simulink model "INS"  (R2018b)
settings: configuration reference "ins_config" (kept outside this file)
values from neighbouring files (symbols this model uses):
  INS_EXPORT = Simulink.Parameter(INS_EXPORT_VALUE)    [ins_model_init.m]
  INS_PARAM = Simulink.Parameter(INS_PARAM_VALUE)    [ins_model_init.m]
undefined symbols (not defined in the file or in its folder): DiscIntNeverNeededParam, INS_CONST, INS_EXPORT_VALUE, Sensor_Meas
libraries: simulink x131, FMT_Model_Lib x48
(part 2 of 6)

== system INS/Sensor_PreProcess/MAG_PreProcess/Mag_Data_Process ==
  mag_B_uT : Inport
  mag_valid : Inport  Port=2
  DCM_OB : Inport  Port=3
  GPS_Data : Inport  Port=4
  Bus Selector : BusSelector  OutputSignals=lat_0_rad,lon_0_rad
  Bus Selector1 : BusSelector  OutputSignals=GPS_valid
  Mag_Quality_Estimate : Subsystem
  WMM_Compensation : Subsystem
  WMM_LUT : Subsystem  mask{wmm_magnitude=INS_CONST.wmm_mag, wmm_declination=INS_CONST.wmm_dec, wmm_inclination=INS_CONST.wmm_inc, resolution=10}
      mask prompts: wmm_magnitude "WMM Magnitude Lookup Table"; wmm_declination "WMM Declination Lookup Table"; wmm_inclination "WMM Inclination Lookup Table"; resolution "Resolution (deg)"
  mag_normalized_B : Outport
  mag_quality : Outport  Port=2
  wires:
  Mag_Quality_Estimate/1(mag_quality) -> mag_quality/1
  WMM_LUT/3(inclination_deg) -> Mag_Quality_Estimate/2(nominal_inc_deg)
  mag_B_uT/1 -> WMM_Compensation/4(mag_B_uT)
  DCM_OB/1 -> WMM_Compensation/3(DCM_OB)
  WMM_Compensation/2(mag_normalized_O) -> Mag_Quality_Estimate/1(mag_normalized_O)
  WMM_LUT/1(magnitude_uT) -> WMM_Compensation/1(WMM_magnitude_uT)
  WMM_LUT/2(declination_deg) -> WMM_Compensation/2(WMM_declination_deg)
  GPS_Data/1 -> Bus Selector1/1, Bus Selector/1
  Bus Selector/1 -> WMM_LUT/1(lat_rad)  "<lat_0_rad>"
  Bus Selector/2 -> WMM_LUT/2(lon_rad)  "<lon_0_rad>"
  Bus Selector1/1 -> Mag_Quality_Estimate/3(pos_0_valid), WMM_Compensation/5(pos_0_valid)  "<GPS_valid>"
  mag_valid/1 -> Mag_Quality_Estimate/4(mag_valid)
  WMM_Compensation/1(mag_normalized_B) -> mag_normalized_B/1

== system INS/Sensor_PreProcess/MAG_PreProcess/Sensor_Valid ==
  mag_B_gauss : Inport
  timestamp_ms : Inport  Port=2
  Compare To Constant4 : simulink/Logic and Bit Operations/Compare To Constant  relop=<  const=timeout  OutDataTypeStr=boolean
  Constant : Constant  Value=INS_EXPORT.period  OutDataTypeStr=single
  Detect Change : simulink/Logic and Bit Operations/Detect Change  vinit=0  OutDataTypeStr=boolean
  Discrete-Time Integrator : DiscreteIntegrator  IntegratorMethod=Accumulation: Forward Euler  ExternalReset=sampled level  SampleTime=-1  OutDataTypeStr=uint32  SaturateOnIntegerOverflow=on  ICPrevOutput=DiscIntNeverNeededParam  ICPrevScaledInput=DiscIntNeverNeededParam
  Ever_Valid : Subsystem
  Interval Test1 : simulink/Logic and Bit Operations/Interval Test  IntervalClosedRight=off  uplimit=mag_max  IntervalClosedLeft=off  lowlimit=mag_min  OutDataTypeStr=boolean
  Logical Operator1 : Logic  Inputs=1  AllPortsSameDT=off  OutDataTypeStr=boolean
  Logical Operator4 : Logic  Inputs=3  AllPortsSameDT=off  OutDataTypeStr=boolean
  valid : Outport
  wires:
  Logical Operator4/1 -> valid/1
  Compare To Constant4/1 -> Logical Operator4/2
  Discrete-Time Integrator/1 -> Compare To Constant4/1
  Detect Change/1 -> Ever_Valid/1(in), Discrete-Time Integrator/2
  Constant/1 -> Discrete-Time Integrator/1
  Logical Operator1/1 -> Logical Operator4/1
  timestamp_ms/1 -> Detect Change/1
  mag_B_gauss/1 -> Interval Test1/1
  Interval Test1/1 -> Logical Operator1/1
  Ever_Valid/1(out) -> Logical Operator4/3

== system INS/Sensor_PreProcess/OpticalFlow_PreProcess/Height_Compensation ==
  OpticalFlow_Bus : Inport
  IMU_Data : Inport  Port=2
  Rangefinder_Data : Inport  Port=3
  Bus Selector : BusSelector  OutputSignals=vx,vy
  Bus Selector1 : BusSelector  OutputSignals=distance,valid
  Bus Selector2 : BusSelector  OutputSignals=gyr_y,gyr_x
  DeadZone : Subsystem  mask{dz=0.5}
      mask prompts: dz "dead zone"
  Demux : Demux  Outputs=2
  First Order LPF : FMT_Model_Lib/Filter/First Order LPF  fc=30
      settings: SourceProductName=FMT Toolbox
  First Order LPF1 : FMT_Model_Lib/Filter/First Order LPF  fc=10
      settings: SourceProductName=FMT Toolbox
  Gain : Gain  Gain=-1
  Gain1 : Gain  Gain=INS_PARAM.OPF_FIX_GAIN
  Multiply : Product  Inputs=3
  Mux : Mux  Inputs=2
  Mux1 : Mux  Inputs=2
  Sum : Sum  Inputs=|+-
  vx_B_mPs : Outport
  vy_B_mPs : Outport  Port=2
  wires:
  Rangefinder_Data/1 -> Bus Selector1/1
  OpticalFlow_Bus/1 -> Bus Selector/1
  Bus Selector/1 -> Mux/1  "<vx>"
  Bus Selector/2 -> Mux/2  "<vy>"
  Bus Selector1/1 -> Multiply/2  "<distance>"
  Mux/1 -> First Order LPF/1
  Demux/1 -> vx_B_mPs/1
  Demux/2 -> vy_B_mPs/1
  First Order LPF/1 -> Sum/1  "raw_vxy"
  Multiply/1 -> Demux/1
  Bus Selector1/2 -> Multiply/3  "<valid>"
  IMU_Data/1 -> Bus Selector2/1
  Bus Selector2/1 -> Mux1/1  "<gyr_y>"
  Bus Selector2/2 -> Gain/1  "<gyr_x>"
  Gain/1 -> Mux1/2
  Mux1/1 -> First Order LPF1/1
  DeadZone/1(y) -> Gain1/1
  Gain1/1 -> Sum/2  "gyro_vxy"
  Sum/1 -> Multiply/1  "fix_vxy"
  First Order LPF1/1 -> DeadZone/1(u)

== system INS/Sensor_PreProcess/OpticalFlow_PreProcess/Sensor_Valid ==
  OpticalFlow_Bus : Inport
  Rangefinder_Data : Inport  Port=2
  Bus Selector : BusSelector  OutputSignals=vx,vy,quality,timestamp
  Bus Selector1 : BusSelector  OutputSignals=valid
  Compare To Constant4 : simulink/Logic and Bit Operations/Compare To Constant  relop=<  const=timeout  OutDataTypeStr=boolean
  Constant : Constant  Value=INS_EXPORT.period  OutDataTypeStr=single
  Detect Change : simulink/Logic and Bit Operations/Detect Change  vinit=0  OutDataTypeStr=boolean
  Discrete-Time Integrator : DiscreteIntegrator  IntegratorMethod=Accumulation: Forward Euler  ExternalReset=sampled level  SampleTime=-1  OutDataTypeStr=uint32  SaturateOnIntegerOverflow=on  ICPrevOutput=DiscIntNeverNeededParam  ICPrevScaledInput=DiscIntNeverNeededParam
  Ever_Valid : Subsystem
  Interval Test1 : simulink/Logic and Bit Operations/Interval Test  IntervalClosedRight=off  uplimit=max_vel  IntervalClosedLeft=off  lowlimit=min_vel  OutDataTypeStr=boolean
  Interval Test2 : simulink/Logic and Bit Operations/Interval Test  IntervalClosedRight=off  uplimit=max_vel  IntervalClosedLeft=off  lowlimit=min_vel  OutDataTypeStr=boolean
  Logical Operator : Logic  AllPortsSameDT=off  OutDataTypeStr=boolean
  Logical Operator1 : Logic  Inputs=5  AllPortsSameDT=off  OutDataTypeStr=boolean
  Relay : Relay  OnOutputValue=q_high  OffOutputValue=q_low
  valid : Outport
  wires:
  Logical Operator1/1 -> valid/1
  Compare To Constant4/1 -> Logical Operator1/3
  Detect Change/1 -> Ever_Valid/1(in), Discrete-Time Integrator/2
  Constant/1 -> Discrete-Time Integrator/1
  Discrete-Time Integrator/1 -> Compare To Constant4/1
  Bus Selector/4 -> Detect Change/1  "<timestamp>"
  OpticalFlow_Bus/1 -> Bus Selector/1
  Bus Selector/1 -> Interval Test1/1  "<vx>"
  Bus Selector/2 -> Interval Test2/1  "<vy>"
  Interval Test1/1 -> Logical Operator/1
  Interval Test2/1 -> Logical Operator/2
  Bus Selector/3 -> Relay/1  "<quality>"
  Logical Operator/1 -> Logical Operator1/1
  Relay/1 -> Logical Operator1/2
  Rangefinder_Data/1 -> Bus Selector1/1
  Bus Selector1/1 -> Logical Operator1/5  "<valid>"
  Ever_Valid/1(out) -> Logical Operator1/4

== system INS/Sensor_PreProcess/Rangefinder_PreProcess/Sensor_Valid ==
  Rangefinder_Bus : Inport
  Bus Selector : BusSelector  OutputSignals=distance,timestamp
  Compare To Constant4 : simulink/Logic and Bit Operations/Compare To Constant  relop=<  const=timeout  OutDataTypeStr=boolean
  Constant : Constant  Value=INS_EXPORT.period  OutDataTypeStr=single
  Detect Change : simulink/Logic and Bit Operations/Detect Change  vinit=0  OutDataTypeStr=boolean
  Discrete-Time Integrator : DiscreteIntegrator  IntegratorMethod=Accumulation: Forward Euler  ExternalReset=sampled level  SampleTime=-1  OutDataTypeStr=uint32  SaturateOnIntegerOverflow=on  ICPrevOutput=DiscIntNeverNeededParam  ICPrevScaledInput=DiscIntNeverNeededParam
  Ever_Valid : Subsystem
  Interval Test3 : simulink/Logic and Bit Operations/Interval Test  IntervalClosedRight=off  uplimit=max_alt  IntervalClosedLeft=off  lowlimit=min_alt  OutDataTypeStr=boolean
  Logical Operator1 : Logic  Inputs=4  AllPortsSameDT=off  OutDataTypeStr=boolean
  Relay : Relay  OnSwitchValue=max_alt  OffSwitchValue=max_alt-(max_alt-min_alt)/4  OnOutputValue=0  OffOutputValue=1
  valid : Outport
  wires:
  Bus Selector/1 -> Interval Test3/1, Relay/1  "<distance>"
  Rangefinder_Bus/1 -> Bus Selector/1
  Bus Selector/2 -> Detect Change/1  "<timestamp>"
  Discrete-Time Integrator/1 -> Compare To Constant4/1
  Constant/1 -> Discrete-Time Integrator/1
  Relay/1 -> Logical Operator1/2
  Compare To Constant4/1 -> Logical Operator1/3
  Logical Operator1/1 -> valid/1
  Detect Change/1 -> Ever_Valid/1(in), Discrete-Time Integrator/2
  Ever_Valid/1(out) -> Logical Operator1/4
  Interval Test3/1 -> Logical Operator1/1

== system INS/Sensor_PreProcess/Rangefinder_PreProcess/Subsystem ==
  in : Inport
  Compare To Constant : simulink/Logic and Bit Operations/Compare To Constant  relop=>=  const=20  OutDataTypeStr=boolean
  Compare To Zero : simulink/Logic and Bit Operations/Compare To Zero  relop=>  OutDataTypeStr=boolean
  Discrete-Time Integrator : DiscreteIntegrator  IntegratorMethod=Accumulation: Forward Euler  ExternalReset=falling  SampleTime=-1  OutDataTypeStr=uint32  LimitOutput=on  UpperSaturationLimit=9999  LowerSaturationLimit=0  ICPrevOutput=DiscIntNeverNeededParam  ICPrevScaledInput=DiscIntNeverNeededParam
  out : Outport
  wires:
  in/1 -> Compare To Zero/1
  Compare To Zero/1 -> Discrete-Time Integrator/2, Discrete-Time Integrator/1
  Discrete-Time Integrator/1 -> Compare To Constant/1
  Compare To Constant/1 -> out/1

== system INS/Sensor_PreProcess/Rangefinder_PreProcess/Tilt_Compensation ==
  Rangefinder_Bus : Inport
  Rotation_Data : Inport  Port=2
  Bus Selector : BusSelector  OutputSignals=distance
  Bus Selector1 : BusSelector  OutputSignals=phi_rad,theta_rad
  Cos : Trigonometry  Operator=cos
  Cos1 : Trigonometry  Operator=cos
  Multiply : Product  Inputs=3
  raw_distance : Outport
  distance : Outport  Port=2
  wires:
  Bus Selector1/1 -> Cos/1  "<phi_rad>"
  Cos/1 -> Multiply/2
  Rangefinder_Bus/1 -> Bus Selector/1
  Multiply/1 -> distance/1
  Bus Selector/1 -> raw_distance/1, Multiply/1  "<distance>"
  Bus Selector1/2 -> Cos1/1  "<theta_rad>"
  Cos1/1 -> Multiply/3
  Rotation_Data/1 -> Bus Selector1/1

== system INS/Bus_Constructor/Status_Output/INS_Flag/INS_Ready ==
  Rotation_Data : Inport
  Bus Selector : BusSelector  OutputSignals=att_reset,heading_reset
  Delay : Delay  DelayLength=1
  Delay1 : Delay  DelayLength=1
  Detect Increase : simulink/Logic and Bit Operations/Detect Increase  vinit=0.0  OutDataTypeStr=boolean
  Detect Increase1 : simulink/Logic and Bit Operations/Detect Increase  vinit=0.0  OutDataTypeStr=boolean
  Logical Operator : Logic  AllPortsSameDT=off  OutDataTypeStr=boolean
  Logical Operator1 : Logic  Operator=OR  AllPortsSameDT=off  OutDataTypeStr=boolean
  Logical Operator2 : Logic  Operator=OR  AllPortsSameDT=off  OutDataTypeStr=boolean
  ready : Outport
  wires:
  Rotation_Data/1 -> Bus Selector/1
  Detect Increase/1 -> Logical Operator1/1
  Logical Operator1/1 -> Logical Operator/1, Delay/1
  Delay/1 -> Logical Operator1/2
  Bus Selector/1 -> Detect Increase/1  "<att_reset>"
  Logical Operator2/1 -> Logical Operator/2, Delay1/1
  Detect Increase1/1 -> Logical Operator2/1
  Delay1/1 -> Logical Operator2/2
  Bus Selector/2 -> Detect Increase1/1  "<heading_reset>"
  Logical Operator/1 -> ready/1

== system INS/Bus_Constructor/Status_Output/INS_Flag/valid_check5 ==
  quality : Inport
  Compare To Constant : simulink/Logic and Bit Operations/Compare To Constant  relop=>=  const=time_out  OutDataTypeStr=boolean
  Compare To Constant1 : simulink/Logic and Bit Operations/Compare To Constant  relop=>  const=0  OutDataTypeStr=boolean
  Compare To Constant2 : simulink/Logic and Bit Operations/Compare To Constant  relop=>  const=0  OutDataTypeStr=boolean
  Constant : Constant  Value=INS_EXPORT.period  OutDataTypeStr=Inherit: Inherit via back propagation
  Delay : Delay  DelayLength=1
  Detect Rise Positive : simulink/Logic and Bit Operations/Detect Rise Positive  vinit=0  OutDataTypeStr=boolean
  Discrete-Time Integrator : DiscreteIntegrator  IntegratorMethod=Accumulation: Forward Euler  gainval=1  ExternalReset=level  SampleTime=-1  LimitOutput=on  UpperSaturationLimit=1e6  LowerSaturationLimit=0  ICPrevOutput=DiscIntNeverNeededParam  ICPrevScaledInput=DiscIntNeverNeededParam
  Logical Operator : Logic  Operator=NOT  AllPortsSameDT=off  OutDataTypeStr=boolean
  Logical Operator1 : Logic  Operator=OR  AllPortsSameDT=off  OutDataTypeStr=boolean
  Multiply : Product
  valid : Outport
  wires:
  Multiply/1 -> valid/1
  Delay/1 -> Multiply/2, Logical Operator1/2
  Logical Operator1/1 -> Delay/1
  Detect Rise Positive/1 -> Logical Operator1/1
  Compare To Constant2/1 -> Detect Rise Positive/1
  quality/1 -> Compare To Constant1/1, Compare To Constant2/1
  Compare To Constant1/1 -> Discrete-Time Integrator/2
  Constant/1 -> Discrete-Time Integrator/1
  Discrete-Time Integrator/1 -> Compare To Constant/1
  Compare To Constant/1 -> Logical Operator/1
  Logical Operator/1 -> Multiply/1

== system INS/Bus_Constructor/Status_Output/INS_Flag/valid_check8 ==
  quality : Inport
  Compare To Constant : simulink/Logic and Bit Operations/Compare To Constant  relop=>=  const=time_out  OutDataTypeStr=boolean
  Compare To Constant1 : simulink/Logic and Bit Operations/Compare To Constant  relop=>  const=0  OutDataTypeStr=boolean
  Compare To Constant2 : simulink/Logic and Bit Operations/Compare To Constant  relop=>  const=0  OutDataTypeStr=boolean
  Constant : Constant  Value=INS_EXPORT.period  OutDataTypeStr=Inherit: Inherit via back propagation
  Delay : Delay  DelayLength=1
  Detect Rise Positive : simulink/Logic and Bit Operations/Detect Rise Positive  vinit=0  OutDataTypeStr=boolean
  Discrete-Time Integrator : DiscreteIntegrator  IntegratorMethod=Accumulation: Forward Euler  gainval=1  ExternalReset=level  SampleTime=-1  LimitOutput=on  UpperSaturationLimit=1e6  LowerSaturationLimit=0  ICPrevOutput=DiscIntNeverNeededParam  ICPrevScaledInput=DiscIntNeverNeededParam
  Logical Operator : Logic  Operator=NOT  AllPortsSameDT=off  OutDataTypeStr=boolean
  Logical Operator1 : Logic  Operator=OR  AllPortsSameDT=off  OutDataTypeStr=boolean
  Multiply : Product
  valid : Outport
  wires:
  Multiply/1 -> valid/1
  Delay/1 -> Multiply/2, Logical Operator1/2
  Logical Operator1/1 -> Delay/1
  Detect Rise Positive/1 -> Logical Operator1/1
  Compare To Constant2/1 -> Detect Rise Positive/1
  quality/1 -> Compare To Constant1/1, Compare To Constant2/1
  Compare To Constant1/1 -> Discrete-Time Integrator/2
  Constant/1 -> Discrete-Time Integrator/1
  Discrete-Time Integrator/1 -> Compare To Constant/1
  Compare To Constant/1 -> Logical Operator/1
  Logical Operator/1 -> Multiply/1

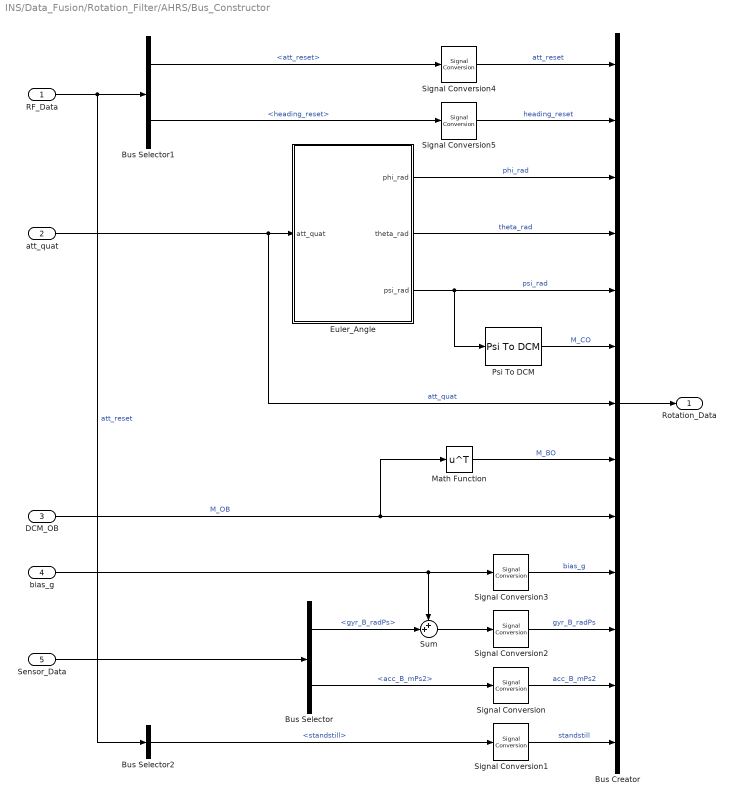
== system INS/Data_Fusion/Rotation_Filter/AHRS/Bus_Constructor ==
  RF_Data : Inport
  att_quat : Inport  Port=2
  DCM_OB : Inport  Port=3
  bias_g : Inport  Port=4
  Sensor_Data : Inport  Port=5
  Bus Creator : BusCreator  Inputs=13
  Bus Selector : BusSelector  OutputSignals=IMU_Data.gyr_B_radPs,IMU_Data.acc_B_mPs2
  Bus Selector1 : BusSelector  OutputSignals=att_reset,heading_reset
  Bus Selector2 : BusSelector  OutputSignals=standstill
  Euler_Angle : Subsystem
  Math Function : Math  Operator=transpose  SaturateOnIntegerOverflow=on
  Psi To DCM : FMT_Model_Lib/Transformation/Psi To DCM
      settings: SourceProductName=FMT Toolbox
  Signal Conversion{,1..5} (6 alike) : SignalConversion  OverrideOpt=off
  Sum : Sum  Inputs=++|
  Rotation_Data : Outport
  wires:
  Bus Selector1/1 -> Signal Conversion4/1  "<att_reset>"
  Signal Conversion/1 -> Bus Creator/12  "acc_B_mPs2"
  Euler_Angle/1(phi_rad) -> Bus Creator/3  "phi_rad"
  Euler_Angle/2(theta_rad) -> Bus Creator/4  "theta_rad"
  Euler_Angle/3(psi_rad) -> Psi To DCM/1, Bus Creator/5  "psi_rad"
  Sensor_Data/1 -> Bus Selector/1
  Bus Selector2/1 -> Signal Conversion1/1  "<standstill>"
  Bus Creator/1 -> Rotation_Data/1
  bias_g/1 -> Sum/1, Signal Conversion3/1
  Math Function/1 -> Bus Creator/8  "M_BO"
  DCM_OB/1 -> Math Function/1, Bus Creator/9  "M_OB"
  att_quat/1 -> Euler_Angle/1(att_quat), Bus Creator/7  "att_quat"
  Psi To DCM/1 -> Bus Creator/6  "M_CO"
  Signal Conversion1/1 -> Bus Creator/13  "standstill"
  Bus Selector/2 -> Signal Conversion/1  "<acc_B_mPs2>"
  Signal Conversion2/1 -> Bus Creator/11  "gyr_B_radPs"
  Signal Conversion3/1 -> Bus Creator/10  "bias_g"
  RF_Data/1 -> Bus Selector2/1, Bus Selector1/1  "att_reset"
  Bus Selector/1 -> Sum/2  "<gyr_B_radPs>"
  Signal Conversion4/1 -> Bus Creator/1  "att_reset"
  Bus Selector1/2 -> Signal Conversion5/1  "<heading_reset>"
  Signal Conversion5/1 -> Bus Creator/2  "heading_reset"
  Sum/1 -> Signal Conversion2/1

== system INS/Data_Fusion/Rotation_Filter/AHRS/Correct ==
  Rotation_Data : Inport
  Translation_Data : Inport  Port=2
  Sensor_Data : Inport  Port=3
  RF_Data : Inport  Port=4
  Attitude_Correction : Subsystem
  Bus Selector1 : BusSelector  OutputSignals=IMU_Data
  Gyro_Bias_Correction : Subsystem
  att_B_correction : Outport
  bias_g_B_correction : Outport  Port=2
  wires:
  Gyro_Bias_Correction/1(bias_g_B_correction) -> bias_g_B_correction/1
  Bus Selector1/1 -> Gyro_Bias_Correction/2(IMU_Data)  "<IMU_Data>"
  RF_Data/1 -> Attitude_Correction/4(RF_Data)
  Attitude_Correction/1(att_B_correction) -> att_B_correction/1, Gyro_Bias_Correction/1(att_B_correction)
  Sensor_Data/1 -> Attitude_Correction/2(Sensor_Data), Bus Selector1/1
  Rotation_Data/1 -> Attitude_Correction/3(Rotation_Data)
  Translation_Data/1 -> Attitude_Correction/1(Translation_Data)

== system INS/Data_Fusion/Rotation_Filter/AHRS/Update ==
  att_B_correction : Inport
  bias_g_correction : Inport  Port=2
  RF_Data : Inport  Port=3
  Sensor_Data : Inport  Port=4
  Attitude_Update : Subsystem
  Attitude_Update1 : Subsystem  Commented=on
  Bus Selector : BusSelector  OutputSignals=IMU_Data.gyr_B_radPs
  Bus Selector1 : BusSelector  OutputSignals=att_reset,quat_0
  Gyro_Bias_Update : Subsystem
  Sum2 : Sum  Inputs=|++
  att_quat : Outport
  DCM_OB : Outport  Port=2
  bias_g : Outport  Port=3
  wires:
  Sensor_Data/1 -> Bus Selector/1
  Gyro_Bias_Update/1(gyr_B_correction) -> Sum2/2
  att_B_correction/1 -> Sum2/1
  Sum2/1 -> Attitude_Update/3(att_B_correction)
  Bus Selector/1 -> Gyro_Bias_Update/2(gyr_B_radPs)  "<gyr_B_radPs>"
  bias_g_correction/1 -> Gyro_Bias_Update/1(bias_g_correction)
  Attitude_Update/1(att_quat) -> att_quat/1
  Attitude_Update/2(DCM_OB) -> DCM_OB/1
  Gyro_Bias_Update/2(bias_g) -> bias_g/1
  RF_Data/1 -> Bus Selector1/1  "att_reset"
  Bus Selector1/1 -> Attitude_Update/1(att_reset)  "<att_reset>"
  Bus Selector1/2 -> Attitude_Update/2(quat_0)  "<quat_0>"

== system INS/Data_Fusion/Rotation_Filter/RF_Data_PreProcess/Attitude_Reset ==
  Sensor_Data : Inport
  Bus Selector : BusSelector  OutputSignals=IMU_Data.IMU_valid,IMU_Data.acc_B_mPs2
  Bus Selector2 : BusSelector  OutputSignals=Mag_Data.mag_quality,Mag_Data.mag_norm_B
  Bus Selector3 : BusSelector  OutputSignals=ExternalPos_Data.heading_valid,GPS_Data.heading_valid
  Compare To Constant : simulink/Logic and Bit Operations/Compare To Constant  relop=>  const=0.01  OutDataTypeStr=boolean
  Compare To Constant1 : simulink/Logic and Bit Operations/Compare To Constant  relop=>=  const=0.2  OutDataTypeStr=boolean
  Detect Rise Positive : simulink/Logic and Bit Operations/Detect Rise Positive  vinit=0  OutDataTypeStr=boolean
  Detect Rise Positive1 : simulink/Logic and Bit Operations/Detect Rise Positive  vinit=0  OutDataTypeStr=boolean
  Interval Test : simulink/Logic and Bit Operations/Interval Test  IntervalClosedRight=on  uplimit=INS_CONST.g+0.5  IntervalClosedLeft=on  lowlimit=INS_CONST.g-0.5  OutDataTypeStr=boolean
  Logical Operator1 : Logic  AllPortsSameDT=off  OutDataTypeStr=boolean
  Logical Operator3 : Logic  AllPortsSameDT=off  OutDataTypeStr=boolean
  Logical Operator4 : Logic  Operator=OR  Inputs=3  AllPortsSameDT=off  OutDataTypeStr=boolean
  Logical Operator5 : Logic  Operator=OR  AllPortsSameDT=off  OutDataTypeStr=boolean
  Vector Modulus : FMT_Model_Lib/Math/Vector Modulus
      settings: SourceProductName=FMT Toolbox
  Vector Modulus1 : FMT_Model_Lib/Math/Vector Modulus
      settings: SourceProductName=FMT Toolbox
  sample_valid : Subsystem
  sample_valid1 : Subsystem
  att_reset : Outport
  heading_reset : Outport  Port=2
  wires:
  sample_valid/1(imu_valid) -> Detect Rise Positive/1  "tt2"
  Vector Modulus1/1 -> Compare To Constant/1
  Interval Test/1 -> Logical Operator1/2
  Vector Modulus/1 -> Interval Test/1
  Logical Operator1/1 -> sample_valid/1(valid)
  Sensor_Data/1 -> Bus Selector2/1, Bus Selector3/1, Bus Selector/1
  Bus Selector/2 -> Vector Modulus/1  "<acc_B_mPs2>"
  Bus Selector/1 -> Logical Operator1/1  "<IMU_valid>"
  Bus Selector2/2 -> Vector Modulus1/1  "<mag_norm_B>"
  Bus Selector2/1 -> Compare To Constant1/1  "<mag_quality>"
  Compare To Constant/1 -> Logical Operator3/2
  Compare To Constant1/1 -> Logical Operator3/1
  Logical Operator3/1 -> sample_valid1/1(valid)
  sample_valid1/1(mag_valid) -> Logical Operator4/1  "tt1"
  Bus Selector3/1 -> Logical Operator4/2  "<heading_valid>"
  Logical Operator4/1 -> Detect Rise Positive1/1
  Detect Rise Positive1/1 -> Logical Operator5/2, heading_reset/1
  Detect Rise Positive/1 -> Logical Operator5/1
  Logical Operator5/1 -> att_reset/1
  Bus Selector3/2 -> Logical Operator4/3  "<heading_valid>"

== system INS/Data_Fusion/Rotation_Filter/RF_Data_PreProcess/Initial_Attitude ==
  Sensor_Data : Inport
  Enable : EnablePort
  Bus Selector : BusSelector  OutputSignals=IMU_Data.acc_B_mPs2
  Cross Product : FMT_Model_Lib/Math/Cross Product
      settings: SourceProductName=FMT Toolbox
  Cross Product1 : FMT_Model_Lib/Math/Cross Product
      settings: SourceProductName=FMT Toolbox
  DCM To Quaternion : FMT_Model_Lib/Quaternion/DCM To Quaternion
      settings: SourceProductName=FMT Toolbox
  Gain : Gain  Gain=-1
  Heading_Vector : Subsystem
  Vector Concatenate : Concatenate  NumInputs=3  Mode=Multidimensional array  ConcatenateDimension=2
  Vector Normalize : FMT_Model_Lib/Math/Vector Normalize
      settings: SourceProductName=FMT Toolbox
  Vector Normalize1 : FMT_Model_Lib/Math/Vector Normalize
      settings: SourceProductName=FMT Toolbox
  Vector Normalize2 : FMT_Model_Lib/Math/Vector Normalize
      settings: SourceProductName=FMT Toolbox
  quat_0 : Outport  InitialOutput=[1; 0; 0; 0]
  wires:
  Gain/1 -> Cross Product/1, Vector Normalize2/1, Cross Product1/2
  Cross Product1/1 -> Vector Normalize/1
  Cross Product/1 -> Vector Normalize1/1, Cross Product1/1
  Vector Normalize1/1 -> Vector Concatenate/2  "DCM_y"
  Vector Normalize/1 -> Vector Concatenate/1  "DCM_x"
  Vector Normalize2/1 -> Vector Concatenate/3  "DCM_z"
  DCM To Quaternion/1 -> quat_0/1
  Sensor_Data/1 -> Bus Selector/1, Heading_Vector/1(Sensor_Data)
  Bus Selector/1 -> Gain/1  "<acc_B_mPs2>"
  Vector Concatenate/1 -> DCM To Quaternion/1  "M_BO"
  Heading_Vector/1(heading_vec) -> Cross Product/2

== system INS/Data_Fusion/Rotation_Filter/RF_Data_PreProcess/Sensor_Select ==
  standstill : Inport
  Sensor_Data : Inport  Port=2
  Bus Selector : BusSelector  OutputSignals=ExternalPos_Data.heading_valid,GPS_Data.heading_valid
  Bus Selector1 : BusSelector  OutputSignals=Mag_Data.mag_valid
  Constant1 : Constant  Value=INS_PARAM.MAG_FLY_EN
  Logical Operator1 : Logic  Operator=NOT  AllPortsSameDT=off  OutDataTypeStr=boolean
  Logical Operator2 : Logic  AllPortsSameDT=off  OutDataTypeStr=boolean
  Logical Operator3 : Logic  Operator=NOT  AllPortsSameDT=off  OutDataTypeStr=boolean
  Logical Operator4 : Logic  Operator=OR  AllPortsSameDT=off  OutDataTypeStr=boolean
  Logical Operator5 : Logic  Inputs=4  AllPortsSameDT=off  OutDataTypeStr=boolean
  ext_psi_enable : Outport
  gps_psi_enable : Outport  Port=2
  mag_enable : Outport  Port=3
  wires:
  Sensor_Data/1 -> Bus Selector/1, Bus Selector1/1
  Bus Selector/1 -> ext_psi_enable/1, Logical Operator3/1  "<heading_valid>"
  Bus Selector1/1 -> Logical Operator5/3  "<mag_valid>"
  Constant1/1 -> Logical Operator4/1
  standstill/1 -> Logical Operator4/2
  Logical Operator5/1 -> mag_enable/1
  Logical Operator3/1 -> Logical Operator2/1, Logical Operator5/1
  Logical Operator4/1 -> Logical Operator5/4
  Logical Operator1/1 -> Logical Operator5/2
  Logical Operator2/1 -> gps_psi_enable/1
  Bus Selector/2 -> Logical Operator1/1, Logical Operator2/2  "<heading_valid>"

== system INS/Data_Fusion/Rotation_Filter/RF_Data_PreProcess/Standstill ==
  IMU_Data : Inport
  Abs : Abs
  Bus Selector : BusSelector  OutputSignals=gyr_B_radPs
  First Order HPF : FMT_Model_Lib/Filter/First Order HPF  fc=1/(2*pi*0.2)
      settings: SourceProductName=FMT Toolbox
  First Order LPF : FMT_Model_Lib/Filter/First Order LPF  fc=1/(2*pi*0.1)
      settings: SourceProductName=FMT Toolbox
  First Order LPF1 : FMT_Model_Lib/Filter/First Order LPF  fc=1/(2*pi*0.05)
      settings: SourceProductName=FMT Toolbox
  MinMax1 : MinMax  Function=max
  Relay : Relay  OnSwitchValue=10e-3  OffSwitchValue=4e-3  OnOutputValue=0  OffOutputValue=1
  Saturation2 : Saturate  UpperLimit=1  LowerLimit=0
  Selector : Selector  InputPortWidth=3  IndexOptions=Index vector (dialog)  Indices=[1 2]  OutputSizes=1
  standstill : Outport
  wires:
  First Order LPF1/1 -> Relay/1
  Relay/1 -> standstill/1
  Saturation2/1 -> First Order LPF1/1
  First Order HPF/1 -> Abs/1
  Selector/1 -> First Order HPF/1
  Abs/1 -> MinMax1/1
  First Order LPF/1 -> Saturation2/1
  MinMax1/1 -> First Order LPF/1
  Bus Selector/1 -> Selector/1  "<gyr_B_radPs>"
  IMU_Data/1 -> Bus Selector/1

== system INS/Data_Fusion/Translation_Filter/CF/Bus_Constructor ==
  TF_Data : Inport
  Horizontal_States : Inport  Port=2
  Verticle_States : Inport  Port=3
  rf_bias : Inport  Port=4
  Bus Creator : BusCreator  Inputs=19
  Bus Selector : BusSelector  OutputSignals=TF_Control.sensor_valid,TF_Control.WGS84_Ref.WGS84_pos_ref.lat_0_rad,TF_Control.WGS84_Ref.WGS84_pos_ref.lon_0_rad,TF_Control.WGS84_Ref.WGS84_pos_ref.h_0_m,TF_Control.WGS84_Ref.WGS84_derivatives_ref.dx_dlat_0,TF_Control.WGS84_Ref.WGS84_derivatives_ref.dy_dlon_0
  Bus_Select : Subsystem
  Constant : Constant  OutDataTypeStr=Inherit: Inherit via back propagation
  Signal Copy{,1..5} (6 alike) : SignalConversion  OverrideOpt=off
  Translation_Data : Outport
  wires:
  Bus Creator/1 -> Translation_Data/1
  Bus_Select/10(vd_mPs) -> Bus Creator/10  "vd_mPs"
  Bus_Select/9(ve_mPs) -> Bus Creator/9  "ve_mPs"
  Bus_Select/8(vn_mPs) -> Bus Creator/8  "vn_mPs"
  Bus_Select/3(h_m) -> Bus Creator/3  "h_m"
  Bus_Select/2(lon_rad) -> Bus Creator/2  "lon_rad"
  Bus_Select/1(lat_rad) -> Bus Creator/1  "lat_rad"
  Bus_Select/11(ba_mPs2) -> Bus Creator/11  "ba_mPs2"
  Verticle_States/1 -> Bus_Select/2(Verticle_States)
  Horizontal_States/1 -> Bus_Select/1(Horizontal_States)
  TF_Data/1 -> Bus Selector/1, Bus_Select/4(TF_Data)
  Constant/1 -> Bus Creator/19  "init_done"
  Bus_Select/7(h_gnd_m) -> Bus Creator/7  "h_gnd_m"
  Bus_Select/6(h_R_m) -> Bus Creator/6  "h_R_m"
  Bus_Select/4(x_R_m) -> Bus Creator/4  "x_R_m"
  Bus_Select/5(y_R_m) -> Bus Creator/5  "y_R_m"
  Bus Selector/1 -> Signal Copy/1  "<sensor_valid>"
  Signal Copy/1 -> Bus Creator/13  "sensor_valid"
  Bus Selector/2 -> Signal Copy1/1  "<lat_0_rad>"
  Bus Selector/3 -> Signal Copy2/1  "<lon_0_rad>"
  Bus Selector/4 -> Signal Copy3/1  "<h_0_m>"
  Signal Copy1/1 -> Bus Creator/14  "lat_0_rad"
  Signal Copy2/1 -> Bus Creator/15  "lon_0_rad"
  Signal Copy3/1 -> Bus Creator/16  "h_0_m"
  rf_bias/1 -> Bus_Select/3(rf_bias)
  Bus Selector/5 -> Signal Copy4/1  "<dx_dlat_0>"
  Signal Copy4/1 -> Bus Creator/17  "dx_dlat"
  Bus Selector/6 -> Signal Copy5/1  "<dy_dlon_0>"
  Signal Copy5/1 -> Bus Creator/18  "dy_dlon"
  Bus_Select/12(TAS_mPs) -> Bus Creator/12  "TAS_mPs"

== system INS/Data_Fusion/Translation_Filter/CF/Horizontal_Filter ==
  TF_Data : Inport
  Rotation_Data : Inport  Port=2
  Correct : Subsystem
  Predict : Subsystem
  Reshape : Reshape  OutputDimensionality=Column vector (2-D)  OutputDimensions=[7,1]
  States : Outport
  wires:
  Predict/1(X_Predict) -> Correct/1(X_Predict)
  Correct/1(X_Next) -> Reshape/1
  Reshape/1 -> Predict/1(X_Prio), States/1
  TF_Data/1 -> Correct/2(TF_Data), Predict/3(TF_Data)
  Rotation_Data/1 -> Predict/2(Rotation_Data)

== system INS/Data_Fusion/Translation_Filter/CF/Verticle_Filter ==
  TF_Data : Inport
  Rotation_Data : Inport  Port=2
  Correct : Subsystem
  Predict : Subsystem
  Reshape : Reshape  OutputDimensionality=Customize  OutputDimensions=[3,1]
  States : Outport
  rf_bias : Outport  Port=2
  wires:
  Predict/1(X_Predict) -> Correct/1(X_Predict)
  Correct/1(X_Next) -> Reshape/1
  Reshape/1 -> Predict/1(X_Prio), States/1
  TF_Data/1 -> Correct/2(TF_Data), Predict/3(TF_Data)
  Rotation_Data/1 -> Predict/2(Rotation_Data)
  Correct/2(rf_bias) -> rf_bias/1

== system INS/Data_Fusion/Translation_Filter/TF_Data_PreProcess/Sensor_Process ==
  Sensor_Data : Inport
  Rotation_Data : Inport  Port=2
  Sensor_Select : Subsystem
  TF_Sensor_Measures : Subsystem
  TF_Sensor_Status : Subsystem
  Sensor_Status : Outport
  Sensor_Meas : Outport  Port=2
  Sensor_Enable : Outport  Port=3
  wires:
  Sensor_Data/1 -> TF_Sensor_Measures/1(Sensor_Data), TF_Sensor_Status/1(Sensor_Data)
  TF_Sensor_Measures/1(Sensor_Meas) -> Sensor_Meas/1
  TF_Sensor_Status/1(Sensor_Status) -> Sensor_Select/1(Sensor_Status), Sensor_Status/1
  Sensor_Select/1(Sensor_Select) -> Sensor_Enable/1  "Sensor_Enable"
  Rotation_Data/1 -> TF_Sensor_Status/2(Rotation_Data), TF_Sensor_Measures/2(Rotation_Data)

== system INS/Data_Fusion/Translation_Filter/TF_Data_PreProcess/TF_Data_Post_Process ==
  U : Inport
  Rotation_Data : Inport  Port=2
  Bus Assignment : BusAssignment  AssignedSignals=Sensor_Meas.GPS_Meas.x_m,Sensor_Meas.GPS_Meas.y_m,Sensor_Meas.GPS_Meas.h_m,Sensor_Meas.GPS_Meas.vn_mPs,Sensor_Meas.GPS_Meas.ve_mPs,Sensor_Meas.GPS_Meas.vd_mPs
  GPS_OFFSET_Compensation : Subsystem
  Y : Outport
  wires:
  U/1 -> GPS_OFFSET_Compensation/1(TF_Data), Bus Assignment/1
  Bus Assignment/1 -> Y/1
  Rotation_Data/1 -> GPS_OFFSET_Compensation/2(Rotation_Data)
  GPS_OFFSET_Compensation/1(x_m) -> Bus Assignment/2
  GPS_OFFSET_Compensation/2(y_m) -> Bus Assignment/3
  GPS_OFFSET_Compensation/3(h_m) -> Bus Assignment/4
  GPS_OFFSET_Compensation/4(vn_mPs) -> Bus Assignment/5
  GPS_OFFSET_Compensation/5(ve_mPs) -> Bus Assignment/6
  GPS_OFFSET_Compensation/6(vd_mPs) -> Bus Assignment/7

== system INS/Data_Fusion/Translation_Filter/TF_Data_PreProcess/Transfer_Filter_Control ==
  Sensor_Enable : Inport
  Sensor_Meas : Inport  Port=2
  Translation_Data : Inport  Port=3
  Bus Creator : BusCreator  Inputs=4
  Filter_Reset : Subsystem
  Sensor_Valid : Subsystem
  WGS84_Reference : Subsystem
  TF_Control : Outport
  wires:
  WGS84_Reference/1(WGS84_Ref) -> Bus Creator/4  "WGS84_Ref"
  Sensor_Meas/1 -> WGS84_Reference/3(Sensor_Meas)
  Filter_Reset/1(pos_reset) -> Bus Creator/1  "pos_reset"
  Sensor_Enable/1 -> Sensor_Valid/1(Sensor_Enable)
  Filter_Reset/2(height_reset) -> Bus Creator/2  "height_reset"
  Bus Creator/1 -> TF_Control/1
  Translation_Data/1 -> WGS84_Reference/2(Translation_Data)
  Sensor_Valid/1(Sensor_Valid) -> WGS84_Reference/1(Sensor_Valid), Bus Creator/3, Filter_Reset/1(Sensor_Valid)  "sensor_valid"

== system INS/Sensor_PreProcess/AirSpeed_Process/Sensor_Valid/Ever_Valid ==
  in : Inport
  Constant1 : Constant  OutDataTypeStr=uint8
  Delay : Delay  DelayLength=1
  Switch : Switch  Criteria=u2 > Threshold
  out : Outport
  wires:
  Constant1/1 -> Switch/1
  Delay/1 -> Switch/3
  in/1 -> Switch/2
  Switch/1 -> out/1, Delay/1

== system INS/Sensor_PreProcess/Baro_PreProcess/Relative_Height/Reference_Height ==
  h_FL_m : Inport
  Enable : EnablePort  StatesWhenEnabling=reset
  Constant1 : Constant  OutDataTypeStr=uint32
  Delay : Delay  DelayLength=1
  Delay1 : Delay  DelayLength=1
  Divide : Product  Inputs=*/
  Saturation1 : Saturate  UpperLimit=10000  LowerLimit=1
  Sum1 : Sum  Inputs=|++  AccumDataTypeStr=uint32  OutDataTypeStr=uint32  RndMeth=Simplest  SaturateOnIntegerOverflow=on
  Sum2 : Sum  Inputs=|++
  h_R_m : Outport
  wires:
  Saturation1/1 -> Divide/2
  Constant1/1 -> Sum1/1
  Sum1/1 -> Delay1/1, Saturation1/1
  Delay1/1 -> Sum1/2
  Sum2/1 -> Delay/1, Divide/1
  Delay/1 -> Sum2/2
  h_FL_m/1 -> Sum2/1
  Divide/1 -> h_R_m/1

== system INS/Sensor_PreProcess/Baro_PreProcess/Relative_Height/Sampling ==
  timestamp : Inport
  data_valid : Inport  Port=2
  Compare To Constant : simulink/Logic and Bit Operations/Compare To Constant  relop=>  const=200  OutDataTypeStr=boolean
  Delay : Delay  DelayLength=1
  Detect Change : simulink/Logic and Bit Operations/Detect Change  vinit=0  OutDataTypeStr=boolean
  Interval Test3 : simulink/Logic and Bit Operations/Interval Test  IntervalClosedRight=off  uplimit=200  IntervalClosedLeft=off  lowlimit=1  OutDataTypeStr=boolean
  Logical Operator5 : Logic  AllPortsSameDT=off  OutDataTypeStr=boolean
  Saturation : Saturate  UpperLimit=10000  LowerLimit=0
  Sum1 : Sum  Inputs=|++  AccumDataTypeStr=uint32  OutDataTypeStr=uint32  RndMeth=Simplest  SaturateOnIntegerOverflow=on
  sampling : Outport
  initialized : Outport  Port=2
  wires:
  Detect Change/1 -> Logical Operator5/1
  Interval Test3/1 -> sampling/1
  Logical Operator5/1 -> Sum1/1
  Delay/1 -> Saturation/1
  timestamp/1 -> Detect Change/1
  data_valid/1 -> Logical Operator5/2
  Sum1/1 -> Interval Test3/1, Compare To Constant/1, Delay/1
  Saturation/1 -> Sum1/2
  Compare To Constant/1 -> initialized/1

== system INS/Sensor_PreProcess/Baro_PreProcess/Sensor_Valid/Ever_Valid ==
  in : Inport
  Constant1 : Constant  OutDataTypeStr=uint8
  Delay : Delay  DelayLength=1
  Switch : Switch  Criteria=u2 > Threshold
  out : Outport
  wires:
  Constant1/1 -> Switch/1
  Delay/1 -> Switch/3
  in/1 -> Switch/2
  Switch/1 -> out/1, Delay/1

== system INS/Sensor_PreProcess/ExternalPos_Process/Sensor_Valid/Ever_Valid ==
  in : Inport
  Constant1 : Constant  OutDataTypeStr=uint8
  Delay : Delay  DelayLength=1
  Switch : Switch  Criteria=u2 > Threshold
  out : Outport
  wires:
  Constant1/1 -> Switch/1
  Delay/1 -> Switch/3
  in/1 -> Switch/2
  Switch/1 -> out/1, Delay/1

== system INS/Sensor_PreProcess/GPS_PreProcess/Data_Scalling/saturation ==
  psi_in : Inport
  Abs : Abs
  Add : Sum  Inputs=-+
  Compare To Constant : simulink/Logic and Bit Operations/Compare To Constant  relop=>  const=pi  OutDataTypeStr=boolean
  Constant : Constant  Value=2*pi  OutDataTypeStr=single
  Constant1 : Constant  Value=2*pi  OutDataTypeStr=single
  Multiply : Product
  Rem : MATLAB Function  TreatAsAtomicUnit=on
  Sign : Signum
  Switch : Switch  Criteria=u2 > Threshold
  psi_rad : Outport
  wires:
  Constant1/1 -> Rem/2(b)
  psi_in/1 -> Rem/1(a)
  Switch/1 -> psi_rad/1
  Sign/1 -> Multiply/2
  Constant/1 -> Multiply/1
  Multiply/1 -> Add/1
  Add/1 -> Switch/1
  Compare To Constant/1 -> Switch/2
  Abs/1 -> Compare To Constant/1
  Rem/1(y) -> Abs/1, Switch/3, Add/2, Sign/1

== system INS/Sensor_PreProcess/GPS_PreProcess/Status_Quality/GPS_Status ==
  note: GPS Status
      | 0: Idle
      | 1: Ready, 3D fix lost
      | 2: Ready, 3D fix
  not_timeout : Inport
  hAcc : Inport  Port=2
  fixtype : Inport  Port=3
  Compare To Constant : simulink/Logic and Bit Operations/Compare To Constant  relop=<  const=5*1e3  OutDataTypeStr=uint8
  Compare To Constant1 : simulink/Logic and Bit Operations/Compare To Constant  relop=>=  const=3  OutDataTypeStr=uint8
  Logical Operator : Logic  Inputs=3  AllPortsSameDT=off  OutDataTypeStr=fixdt(0,8)
  Logical Operator1 : Logic  Inputs=3  AllPortsSameDT=off  OutDataTypeStr=fixdt(0,8)
  Ready : Subsystem
  Sum1 : Sum  Inputs=|++
  status : Outport
  wires:
  not_timeout/1 -> Logical Operator/3, Logical Operator1/3
  Sum1/1 -> status/1
  Logical Operator1/1 -> Sum1/2  "3D Fix"
  hAcc/1 -> Compare To Constant/1
  Compare To Constant/1 -> Logical Operator/1
  Compare To Constant1/1 -> Logical Operator1/2, Logical Operator/2  "3D Fix"
  fixtype/1 -> Compare To Constant1/1
  Ready/1(ready) -> Sum1/1, Logical Operator1/1  "ready"
  Logical Operator/1 -> Ready/1(valid)

== system INS/Sensor_PreProcess/GPS_PreProcess/Status_Quality/check_timeout ==
  timestamp : Inport
  Compare To Constant4 : simulink/Logic and Bit Operations/Compare To Constant  relop=<  const=500  OutDataTypeStr=boolean
  Constant : Constant  Value=INS_EXPORT.period  OutDataTypeStr=single
  Detect Change : simulink/Logic and Bit Operations/Detect Change  vinit=0  OutDataTypeStr=boolean
  Discrete-Time Integrator : DiscreteIntegrator  IntegratorMethod=Accumulation: Forward Euler  ExternalReset=sampled level  SampleTime=-1  OutDataTypeStr=uint32  SaturateOnIntegerOverflow=on  UpperSaturationLimit=10000  LowerSaturationLimit=0  ICPrevOutput=DiscIntNeverNeededParam  ICPrevScaledInput=DiscIntNeverNeededParam
  valid : Outport
  wires:
  Constant/1 -> Discrete-Time Integrator/1
  timestamp/1 -> Detect Change/1
  Detect Change/1 -> Discrete-Time Integrator/2
  Discrete-Time Integrator/1 -> Compare To Constant4/1
  Compare To Constant4/1 -> valid/1

== system INS/Sensor_PreProcess/GPS_PreProcess/Status_Quality/gps_heading_valid ==
  pos_quality : Inport
  yaw_quality : Inport  Port=2
  Constant2 : Constant  Value=INS_PARAM.GPS_YAW_EN
  Logical Operator : Logic  Inputs=3  AllPortsSameDT=off  OutDataTypeStr=boolean
  Relay1 : Relay  OnSwitchValue=0.7  OffSwitchValue=0.5
  Relay2 : Relay  OnSwitchValue=0.7  OffSwitchValue=0.5
  valid : Outport
  wires:
  Constant2/1 -> Logical Operator/3
  Relay1/1 -> Logical Operator/1
  yaw_quality/1 -> Relay2/1
  Relay2/1 -> Logical Operator/2
  Logical Operator/1 -> valid/1
  pos_quality/1 -> Relay1/1

== system INS/Sensor_PreProcess/GPS_PreProcess/Status_Quality/heading_acc ==
  cAcc : Inport
  Constant7 : Constant  Value=2*pi  OutDataTypeStr=Inherit: Inherit via back propagation
  Gain3 : Gain  Gain=1/(2*pi)  OutDataTypeStr=single
  Gain5 : Gain  Gain=1e-3  OutDataTypeStr=single
  Saturation : Saturate  UpperLimit=1  LowerLimit=0
  Second Order LPF : FMT_Model_Lib/Filter/Second Order LPF  fc=1  zeta=0.707
      settings: SourceProductName=FMT Toolbox
  Sum : Sum  Inputs=+-|
  heading_quality : Outport
  wires:
  Gain5/1 -> Sum/2
  Sum/1 -> Gain3/1
  cAcc/1 -> Gain5/1
  Constant7/1 -> Sum/1
  Saturation/1 -> Second Order LPF/1
  Gain3/1 -> Saturation/1
  Second Order LPF/1 -> heading_quality/1

== system INS/Sensor_PreProcess/GPS_PreProcess/Status_Quality/horizontal_quality ==
  hAcc : Inport
  Constant1 : Constant  Value=INS_PARAM.GPS_HOR_Q_BIAS  OutDataTypeStr=Inherit: Inherit via back propagation
  Gain1 : Gain  Gain=1e-3  OutDataTypeStr=single
  Gain2 : Gain  Gain=INS_PARAM.GPS_HOR_Q_SCALE  OutDataTypeStr=single
  Saturation1 : Saturate  UpperLimit=1  LowerLimit=0
  Second Order LPF : FMT_Model_Lib/Filter/Second Order LPF  fc=1  zeta=0.707
      settings: SourceProductName=FMT Toolbox
  Sum1 : Sum  Inputs=+-|
  hor_quality : Outport
  wires:
  Sum1/1 -> Gain2/1
  Gain1/1 -> Sum1/2  "hAcc_m"
  hAcc/1 -> Gain1/1
  Constant1/1 -> Sum1/1
  Saturation1/1 -> Second Order LPF/1
  Gain2/1 -> Saturation1/1
  Second Order LPF/1 -> hor_quality/1

== system INS/Sensor_PreProcess/GPS_PreProcess/Status_Quality/speed_acc ==
  sAcc : Inport
  Constant7 : Constant  Value=INS_PARAM.GPS_VEL_Q_BIAS  OutDataTypeStr=Inherit: Inherit via back propagation
  Gain3 : Gain  Gain=INS_PARAM.GPS_VEL_Q_SCALE  OutDataTypeStr=single
  Gain5 : Gain  Gain=1e-3  OutDataTypeStr=single
  Saturation : Saturate  UpperLimit=1  LowerLimit=0
  Second Order LPF : FMT_Model_Lib/Filter/Second Order LPF  fc=1  zeta=0.707
      settings: SourceProductName=FMT Toolbox
  Sum : Sum  Inputs=+-|
  spd_quality : Outport
  wires:
  Gain5/1 -> Sum/2  "sAcc_m"
  Sum/1 -> Gain3/1
  sAcc/1 -> Gain5/1
  Constant7/1 -> Sum/1
  Saturation/1 -> Second Order LPF/1
  Gain3/1 -> Saturation/1
  Second Order LPF/1 -> spd_quality/1

== system INS/Sensor_PreProcess/GPS_PreProcess/Status_Quality/vertical_quality ==
  vAcc : Inport
  Constant1 : Constant  Value=INS_PARAM.GPS_VER_Q_BIAS  OutDataTypeStr=Inherit: Inherit via back propagation
  Gain1 : Gain  Gain=1e-3  OutDataTypeStr=single
  Gain2 : Gain  Gain=INS_PARAM.GPS_VER_Q_SCALE  OutDataTypeStr=single
  Saturation1 : Saturate  UpperLimit=1  LowerLimit=0
  Second Order LPF : FMT_Model_Lib/Filter/Second Order LPF  fc=1  zeta=0.707
      settings: SourceProductName=FMT Toolbox
  Sum1 : Sum  Inputs=+-|
  ver_quality : Outport
  wires:
  Sum1/1 -> Gain2/1
  Gain1/1 -> Sum1/2  "vAcc_m"
  vAcc/1 -> Gain1/1
  Constant1/1 -> Sum1/1
  Saturation1/1 -> Second Order LPF/1
  Gain2/1 -> Saturation1/1
  Second Order LPF/1 -> ver_quality/1

== system INS/Sensor_PreProcess/IMU_PreProcess/Sensor_Valid/Ever_Valid ==
  in : Inport
  Constant1 : Constant  OutDataTypeStr=uint8
  Delay : Delay  DelayLength=1
  Switch : Switch  Criteria=u2 > Threshold
  out : Outport
  wires:
  Constant1/1 -> Switch/1
  Delay/1 -> Switch/3
  in/1 -> Switch/2
  Switch/1 -> out/1, Delay/1

== system INS/Sensor_PreProcess/MAG_PreProcess/Mag_Data_Process/Mag_Quality_Estimate ==
  note: TODO: improve this
  mag_normalized_O : Inport
  nominal_inc_deg : Inport  Port=2
  pos_0_valid : Inport  Port=3
  mag_valid : Inport  Port=4
  Data Type Conversion : DataTypeConversion  OutDataTypeStr=single
  Mag_Quality : Subsystem
  Multiply : Product  OutDataTypeStr=Inherit: Same as first input
  Switch : Switch  Criteria=u2 > Threshold
  default_mag_quality : Constant  Value=0.5  OutDataTypeStr=single
  mag_quality : Outport
  wires:
  pos_0_valid/1 -> Switch/2
  default_mag_quality/1 -> Switch/3
  mag_valid/1 -> Multiply/2
  Switch/1 -> Data Type Conversion/1
  Multiply/1 -> mag_quality/1
  nominal_inc_deg/1 -> Mag_Quality/1(nominal_inc_deg)
  mag_normalized_O/1 -> Mag_Quality/2(mag_normalized_O)
  Mag_Quality/1(mag_quality) -> Switch/1
  Data Type Conversion/1 -> Multiply/1

== system INS/Sensor_PreProcess/MAG_PreProcess/Mag_Data_Process/WMM_Compensation ==
  WMM_magnitude_uT : Inport
  WMM_declination_deg : Inport  Port=2
  DCM_OB : Inport  Port=3
  mag_B_uT : Inport  Port=4
  pos_0_valid : Inport  Port=5
  Gain : Gain  Gain=-pi/180  OutDataTypeStr=single
  Math Function2 : Math  Operator=transpose  SaturateOnIntegerOverflow=on
  Product{5..8} (4 alike) : Product  Multiplication=Matrix(*)
  Rotation Matrix Z : FMT_Model_Lib/Transformation/Rotation Matrix Z
      settings: SourceProductName=FMT Toolbox
  Switch3 : Switch  Criteria=u2 > Threshold
  Vector Normalize : FMT_Model_Lib/Math/Vector Normalize
      settings: SourceProductName=FMT Toolbox
  safe_divide : Subsystem
      mask Display:
      | port_label('input', 1, 'x', 'texmode', 'on')
      | port_label('input', 2, '÷', 'texmode', 'on')
  mag_normalized_B : Outport
  mag_normalized_O : Outport  Port=2
  wires:
  Gain/1 -> Rotation Matrix Z/1  "dec_rad"
  WMM_declination_deg/1 -> Gain/1
  mag_B_uT/1 -> Vector Normalize/1, safe_divide/1(u1)  "uT"
  WMM_magnitude_uT/1 -> safe_divide/2(u2)
  safe_divide/1(y) -> Product5/2  "mag_normalized_B"
  DCM_OB/1 -> Product5/1, Math Function2/1, Product7/1
  Product5/1 -> Product6/2  "mag_normalized_O"
  Rotation Matrix Z/1 -> Product6/1
  Product6/1 -> Switch3/1  "mag_norminal_O"
  Math Function2/1 -> Product8/1  "DCM_BO"
  pos_0_valid/1 -> Switch3/2
  Product8/1 -> mag_normalized_B/1
  Switch3/1 -> mag_normalized_O/1, Product8/2
  Vector Normalize/1 -> Product7/2
  Product7/1 -> Switch3/3

== system INS/Sensor_PreProcess/MAG_PreProcess/Mag_Data_Process/WMM_LUT ==
  lat_rad : Inport
  lon_rad : Inport  Port=2
  Add : Sum
  Declination_Lookup_Table : LookupNDDirect  Table=wmm_declination  DiagnosticForOutOfRangeInput=Error
  Demux : Demux  Outputs=2
  Inclination_Lookup_Table : LookupNDDirect  Table=wmm_inclination  DiagnosticForOutOfRangeInput=Error
  Magnitude_Lookup_Table : LookupNDDirect  Table=wmm_magnitude  DiagnosticForOutOfRangeInput=Error
  Mux : Mux  Inputs=2
  Saturation1 : Saturate  UpperLimit=size(wmm_magnitude)-1  LowerLimit=0
  offset : Constant  Value=(size(wmm_magnitude)-1)/2  OutDataTypeStr=int32
  rad_to_index : Gain  Gain=180/pi/resolution  OutDataTypeStr=int32
  magnitude_uT : Outport
  declination_deg : Outport  Port=2
  inclination_deg : Outport  Port=3
  wires:
  Inclination_Lookup_Table/1 -> inclination_deg/1
  Declination_Lookup_Table/1 -> declination_deg/1
  Magnitude_Lookup_Table/1 -> magnitude_uT/1
  offset/1 -> Add/2
  Add/1 -> Saturation1/1
  rad_to_index/1 -> Add/1
  lat_rad/1 -> Mux/1
  lon_rad/1 -> Mux/2
  Mux/1 -> rad_to_index/1
  Saturation1/1 -> Demux/1
  Demux/1 -> Magnitude_Lookup_Table/1, Inclination_Lookup_Table/1, Declination_Lookup_Table/1
  Demux/2 -> Inclination_Lookup_Table/2, Magnitude_Lookup_Table/2, Declination_Lookup_Table/2

== system INS/Sensor_PreProcess/MAG_PreProcess/Sensor_Valid/Ever_Valid ==
  in : Inport
  Constant1 : Constant  OutDataTypeStr=uint8
  Delay : Delay  DelayLength=1
  Switch : Switch  Criteria=u2 > Threshold
  out : Outport
  wires:
  Constant1/1 -> Switch/1
  Delay/1 -> Switch/3
  in/1 -> Switch/2
  Switch/1 -> out/1, Delay/1

== system INS/Sensor_PreProcess/OpticalFlow_PreProcess/Height_Compensation/DeadZone ==
  u : Inport
  Compare To Zero : simulink/Logic and Bit Operations/Compare To Zero  relop=~=  OutDataTypeStr=boolean
  Dead Zone : DeadZone  LowerValue=-dz  UpperValue=dz  SaturateOnIntegerOverflow=on
  Gain : Gain  Gain=dz
  Multiply : Product
  Sign : Signum
  Sum : Sum  Inputs=|++
  y : Outport
  wires:
  u/1 -> Sign/1, Dead Zone/1
  Compare To Zero/1 -> Multiply/1
  Sign/1 -> Gain/1
  Dead Zone/1 -> Compare To Zero/1, Sum/1
  Multiply/1 -> Sum/2
  Sum/1 -> y/1
  Gain/1 -> Multiply/2

== system INS/Sensor_PreProcess/OpticalFlow_PreProcess/Sensor_Valid/Ever_Valid ==
  in : Inport
  Constant1 : Constant  OutDataTypeStr=uint8
  Delay : Delay  DelayLength=1
  Switch : Switch  Criteria=u2 > Threshold
  out : Outport
  wires:
  Constant1/1 -> Switch/1
  Delay/1 -> Switch/3
  in/1 -> Switch/2
  Switch/1 -> out/1, Delay/1

== system INS/Sensor_PreProcess/Rangefinder_PreProcess/Sensor_Valid/Ever_Valid ==
  in : Inport
  Constant1 : Constant  OutDataTypeStr=uint8
  Delay : Delay  DelayLength=1
  Switch : Switch  Criteria=u2 > Threshold
  out : Outport
  wires:
  Constant1/1 -> Switch/1
  Delay/1 -> Switch/3
  in/1 -> Switch/2
  Switch/1 -> out/1, Delay/1

== system INS/Data_Fusion/Rotation_Filter/AHRS/Bus_Constructor/Euler_Angle ==
  att_quat : Inport
  Demux : Demux  Outputs=3
  Quaternion To Euler : FMT_Model_Lib/Quaternion/Quaternion To Euler
      settings: SourceProductName=FMT Toolbox
  phi_rad : Outport
  theta_rad : Outport  Port=2
  psi_rad : Outport  Port=3
  wires:
  Demux/1 -> phi_rad/1
  Demux/2 -> theta_rad/1
  Demux/3 -> psi_rad/1
  att_quat/1 -> Quaternion To Euler/1
  Quaternion To Euler/1 -> Demux/1

== system INS/Data_Fusion/Rotation_Filter/AHRS/Correct/Attitude_Correction ==
  Translation_Data : Inport
  Sensor_Data : Inport  Port=2
  Rotation_Data : Inport  Port=3
  RF_Data : Inport  Port=4
  Attitude_Correct : Subsystem
  Bus Selector2 : BusSelector  OutputSignals=M_BO
  ExternalPsi_Correct : Subsystem
  GPS_Heading_Correct : Subsystem
  Mag_Correct : Subsystem
  Multiply : Product  Multiplication=Matrix(*)
  Sum : Sum  Inputs=|++
  Sum1 : Sum  Inputs=++|
  Sum2 : Sum  Inputs=++|
  att_B_correction : Outport
  wires:
  RF_Data/1 -> Attitude_Correct/3(RF_Data), GPS_Heading_Correct/1(RF_Data), ExternalPsi_Correct/1(RF_Data), Mag_Correct/3(RF_Data)
  Sensor_Data/1 -> GPS_Heading_Correct/3(Sensor_Data), ExternalPsi_Correct/3(Sensor_Data), Mag_Correct/2(Sensor_Data), Attitude_Correct/2(Sensor_Data)
  Attitude_Correct/1(att_corr_O) -> Sum/1  "att_corr_O"
  Multiply/1 -> att_B_correction/1
  Rotation_Data/1 -> GPS_Heading_Correct/2(Rotation_Data), ExternalPsi_Correct/2(Rotation_Data), Mag_Correct/1(Rotation_Data), Bus Selector2/1, Attitude_Correct/1(Rotation_Data)
  Sum/1 -> Multiply/2
  Bus Selector2/1 -> Multiply/1  "<M_BO>"
  Mag_Correct/1(mag_corr_O) -> Sum1/1  "mag_corr_O"
  Sum1/1 -> Sum/2
  Translation_Data/1 -> Mag_Correct/4(Translation_Data)
  ExternalPsi_Correct/1(att_corr_O) -> Sum2/1  "extpsi_corr_O"
  GPS_Heading_Correct/1(att_corr_O) -> Sum2/2  "gps_corr_O"
  Sum2/1 -> Sum1/2
